simulink model "NearSpace_CMG_AttitudeValidation_S03_pitch45"  (R2024a)
settings: Solver=ode4  StartTime=0.0  StopTime=60  FixedStep=.001  RelTol=1e-3
InitFcn:
  | init_paths;
model workspace (MAT data in the model file):
  disturbance_schedule = [0 0.2 0.4 0.6 0.8 1 1.2 1.4 1.6 1.8 2 2.2 ... (1204 elements, 301x4)]
  native_controller_template : object (value not decoded)
  native_reference_bank : object (value not decoded)
  reference_attitude_deg = [0 0.2 0.4 0.6 0.8 1 1.2 1.4 1.6 1.8 2 2.2 ... (1204 elements, 301x4)]
  reference_body_rate = [0 0.2 0.4 0.6 0.8 1 1.2 1.4 1.6 1.8 2 2.2 ... (1204 elements, 301x4)]
  reference_torque_nom = [0 0.2 0.4 0.6 0.8 1 1.2 1.4 1.6 1.8 2 2.2 ... (1204 elements, 301x4)]
  reference_window = [-1e-06 0.199999 0.399999 0.599999 0.799999 0.999999 1.199999 1.399999 1.599999 1.799999 1.999999 2.199999 ... (130032 elements, 301x432)]
libraries: aerolibprivatev1p5 x1
(part 2 of 2)

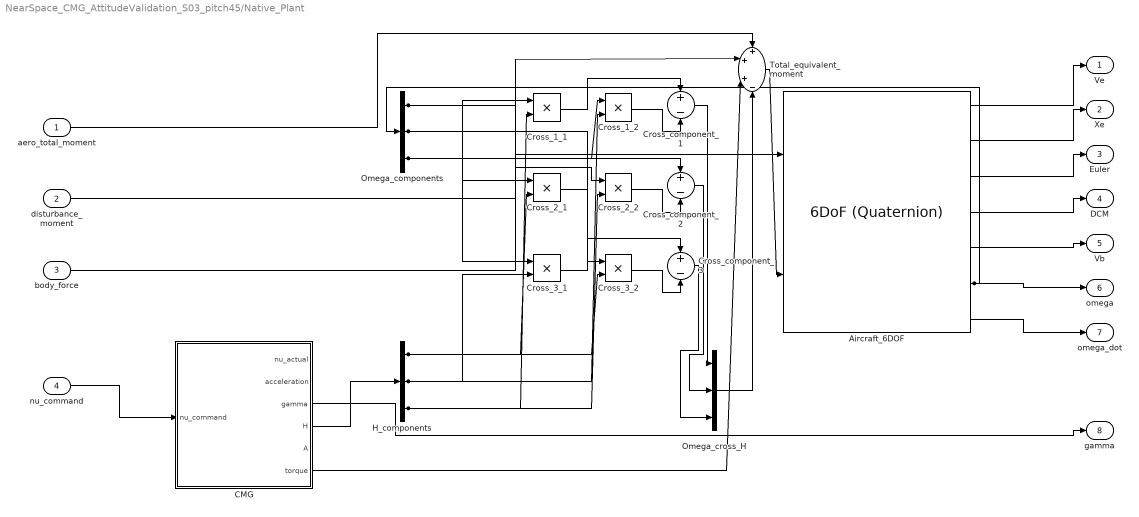
== system NearSpace_CMG_AttitudeValidation_S03_pitch45/Native_Plant ==
  aero_total_moment : Inport  PortDimensions=3
  disturbance_moment : Inport  Port=2  PortDimensions=3
  body_force : Inport  Port=3  PortDimensions=3
  nu_command : Inport  Port=4  PortDimensions=4
  Aircraft_6DOF : aerolibprivatev1p5/6DoF (Quaternion)  xme_0=[0 0 0]  Vm_0=[0 0 0]  eul_0=[-1.7740922954857791e-18;0.21106173041320209;0.087266462599716474]  pm_0=[0 -0.0043273206504133811 -6.9388939039072284e-15]  Mass=1200  Inertia=[1200 0 0;0 8500 0;0 0 9000]  k_quat=1.0
  CMG : Subsystem
  Cross_1_1 : Product
  Cross_1_2 : Product
  Cross_2_1 : Product
  Cross_2_2 : Product
  Cross_3_1 : Product
  Cross_3_2 : Product
  Cross_component_1 : Sum  Inputs=+-
  Cross_component_2 : Sum  Inputs=+-
  Cross_component_3 : Sum  Inputs=+-
  H_components : Demux  Outputs=3
  Omega_components : Demux  Outputs=3
  Omega_cross_H : Mux  Inputs=3
  Total_equivalent_moment : Sum  Inputs=+++-
  Ve : Outport
  Xe : Outport  Port=2
  Euler : Outport  Port=3
  DCM : Outport  Port=4
  Vb : Outport  Port=5
  omega : Outport  Port=6
  omega_dot : Outport  Port=7
  gamma : Outport  Port=8
  wires:
  nu_command/1 -> CMG/1(nu_command)
  Aircraft_6DOF/6 -> omega/1, Omega_components/1
  CMG/4(H) -> H_components/1
  Omega_components/2 -> Cross_3_2/1, Cross_1_1/1
  H_components/3 -> Cross_2_2/2, Cross_1_1/2
  Omega_components/3 -> Cross_2_1/1, Cross_1_2/1
  H_components/2 -> Cross_3_1/2, Cross_1_2/2
  Cross_1_1/1 -> Cross_component_1/1
  Cross_1_2/1 -> Cross_component_1/2
  H_components/1 -> Cross_3_2/2, Cross_2_1/2
  Omega_components/1 -> Cross_3_1/1, Cross_2_2/1
  Cross_2_1/1 -> Cross_component_2/1
  Cross_2_2/1 -> Cross_component_2/2
  Cross_3_1/1 -> Cross_component_3/1
  Cross_3_2/1 -> Cross_component_3/2
  Cross_component_1/1 -> Omega_cross_H/1
  Cross_component_2/1 -> Omega_cross_H/2
  Cross_component_3/1 -> Omega_cross_H/3
  aero_total_moment/1 -> Total_equivalent_moment/1
  disturbance_moment/1 -> Total_equivalent_moment/2
  CMG/6(torque) -> Total_equivalent_moment/3
  Omega_cross_H/1 -> Total_equivalent_moment/4
  Total_equivalent_moment/1 -> Aircraft_6DOF/2
  body_force/1 -> Aircraft_6DOF/1
  Aircraft_6DOF/1 -> Ve/1
  Aircraft_6DOF/2 -> Xe/1
  Aircraft_6DOF/3 -> Euler/1
  Aircraft_6DOF/4 -> DCM/1
  Aircraft_6DOF/5 -> Vb/1
  Aircraft_6DOF/7 -> omega_dot/1
  CMG/3(gamma) -> gamma/1

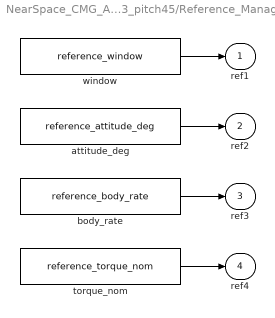
== system NearSpace_CMG_AttitudeValidation_S03_pitch45/Reference_Manager ==
  attitude_deg : FromWorkspace  VariableName=reference_attitude_deg  Interpolate=off  OutputAfterFinalValue=Holding final value
  body_rate : FromWorkspace  VariableName=reference_body_rate  Interpolate=off  OutputAfterFinalValue=Holding final value
  torque_nom : FromWorkspace  VariableName=reference_torque_nom  Interpolate=off  OutputAfterFinalValue=Holding final value
  window : FromWorkspace  VariableName=reference_window  Interpolate=off  OutputAfterFinalValue=Holding final value
  ref1 : Outport
  ref2 : Outport  Port=2
  ref3 : Outport  Port=3
  ref4 : Outport  Port=4
  wires:
  window/1 -> ref1/1
  attitude_deg/1 -> ref2/1
  body_rate/1 -> ref3/1
  torque_nom/1 -> ref4/1

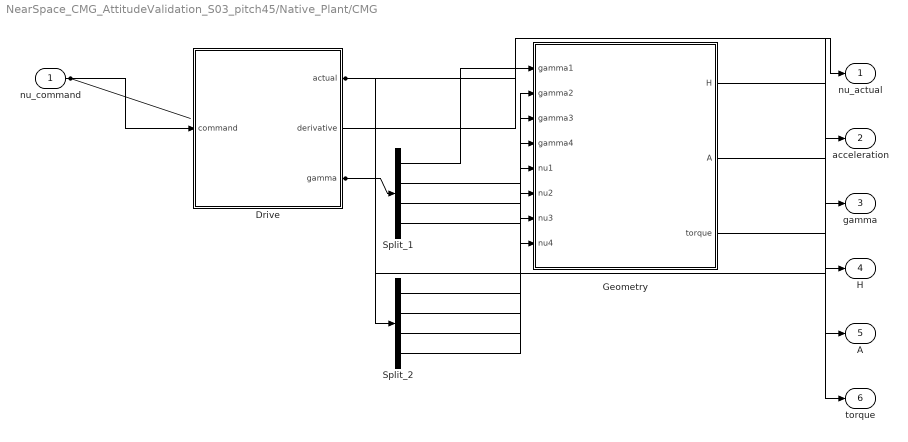
== system NearSpace_CMG_AttitudeValidation_S03_pitch45/Native_Plant/CMG ==
  nu_command : Inport  PortDimensions=4
  Drive : Subsystem
  Geometry : Subsystem
  Split_1 : Demux
  Split_2 : Demux
  nu_actual : Outport
  acceleration : Outport  Port=2
  gamma : Outport  Port=3
  H : Outport  Port=4
  A : Outport  Port=5
  torque : Outport  Port=6
  wires:
  Geometry/3(torque) -> torque/1
  Geometry/2(A) -> A/1
  Geometry/1(H) -> H/1
  Split_2/4 -> Geometry/8(nu4)
  Split_2/3 -> Geometry/7(nu3)
  Split_2/2 -> Geometry/6(nu2)
  Split_2/1 -> Geometry/5(nu1)
  Split_1/4 -> Geometry/4(gamma4)
  Split_1/3 -> Geometry/3(gamma3)
  Split_1/2 -> Geometry/2(gamma2)
  Split_1/1 -> Geometry/1(gamma1)
  nu_command/1 -> Drive/1(command)
  Drive/1(actual) -> Split_2/1, nu_actual/1
  Drive/2(derivative) -> acceleration/1
  Drive/3(gamma) -> Split_1/1, gamma/1

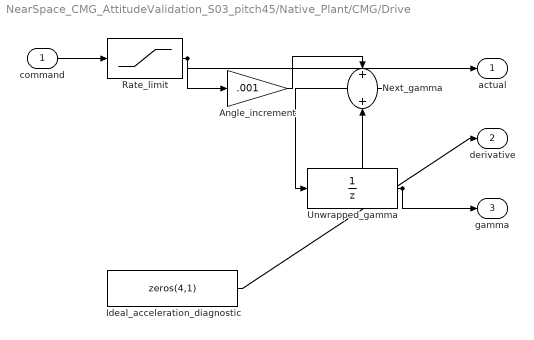
== system NearSpace_CMG_AttitudeValidation_S03_pitch45/Native_Plant/CMG/Drive ==
  command : Inport  PortDimensions=4
  Angle_increment : Gain  Gain=.001
  Ideal_acceleration_diagnostic : Constant  Value=zeros(4,1)
  Next_gamma : Sum
  Rate_limit : Saturate  UpperLimit=1  LowerLimit=-1
  Unwrapped_gamma : UnitDelay  InitialCondition=[0 0 0 0]  SampleTime=.001
  actual : Outport
  derivative : Outport  Port=2
  gamma : Outport  Port=3
  wires:
  command/1 -> Rate_limit/1
  Rate_limit/1 -> actual/1, Angle_increment/1
  Angle_increment/1 -> Next_gamma/1
  Unwrapped_gamma/1 -> Next_gamma/2, gamma/1
  Next_gamma/1 -> Unwrapped_gamma/1
  Ideal_acceleration_diagnostic/1 -> derivative/1

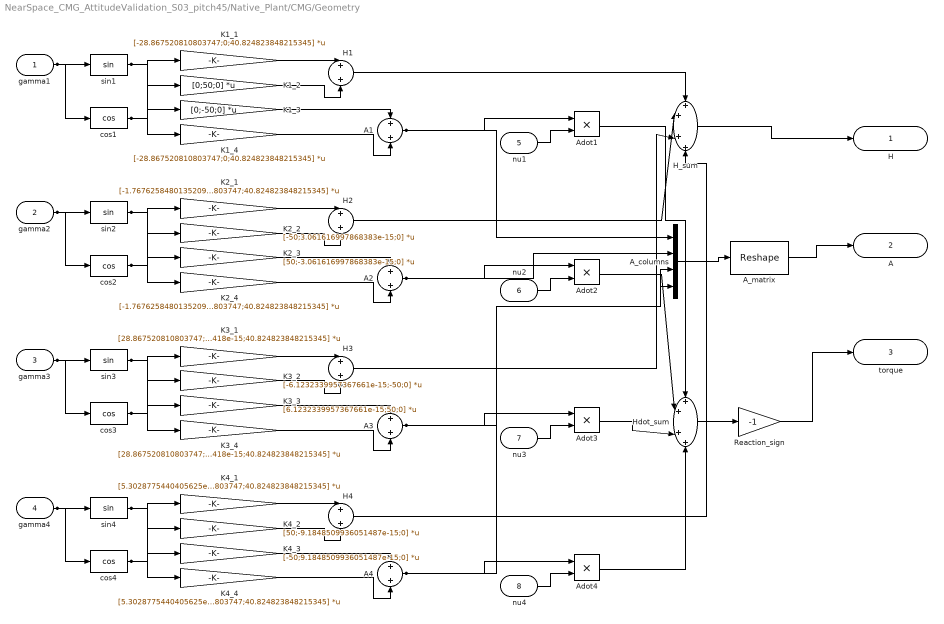
== system NearSpace_CMG_AttitudeValidation_S03_pitch45/Native_Plant/CMG/Geometry ==
  gamma1 : Inport
  gamma2 : Inport  Port=2
  gamma3 : Inport  Port=3
  gamma4 : Inport  Port=4
  nu1 : Inport  Port=5
  nu2 : Inport  Port=6
  nu3 : Inport  Port=7
  nu4 : Inport  Port=8
  A{1..4} (4 alike) : Sum
  A_columns : Mux
  A_matrix : Reshape  OutputDimensionality=Customize  OutputDimensions=[3 4]
  Adot{1..4} (4 alike) : Product
  H{1..4} (4 alike) : Sum
  H_sum : Sum  Inputs=++++
  Hdot_sum : Sum  Inputs=++++
  K1_1 : Gain  Gain=[-28.867520810803747;0;40.824823848215345]  Multiplication=Matrix(K*u)
  K1_2 : Gain  Gain=[0;50;0]  Multiplication=Matrix(K*u)
  K1_3 : Gain  Gain=[0;-50;0]  Multiplication=Matrix(K*u)
  K1_4 : Gain  Gain=[-28.867520810803747;0;40.824823848215345]  Multiplication=Matrix(K*u)
  K2_1 : Gain  Gain=[-1.7676258480135209e-15;-28.867520810803747;40.824823848215345]  Multiplication=Matrix(K*u)
  K2_2 : Gain  Gain=[-50;3.061616997868383e-15;0]  Multiplication=Matrix(K*u)
  K2_3 : Gain  Gain=[50;-3.061616997868383e-15;0]  Multiplication=Matrix(K*u)
  K2_4 : Gain  Gain=[-1.7676258480135209e-15;-28.867520810803747;40.824823848215345]  Multiplication=Matrix(K*u)
  K3_1 : Gain  Gain=[28.867520810803747;-3.5352516960270418e-15;40.824823848215345]  Multiplication=Matrix(K*u)
  K3_2 : Gain  Gain=[-6.1232339957367661e-15;-50;0]  Multiplication=Matrix(K*u)
  K3_3 : Gain  Gain=[6.1232339957367661e-15;50;0]  Multiplication=Matrix(K*u)
  K3_4 : Gain  Gain=[28.867520810803747;-3.5352516960270418e-15;40.824823848215345]  Multiplication=Matrix(K*u)
  K4_1 : Gain  Gain=[5.3028775440405625e-15;28.867520810803747;40.824823848215345]  Multiplication=Matrix(K*u)
  K4_2 : Gain  Gain=[50;-9.1848509936051487e-15;0]  Multiplication=Matrix(K*u)
  K4_3 : Gain  Gain=[-50;9.1848509936051487e-15;0]  Multiplication=Matrix(K*u)
  K4_4 : Gain  Gain=[5.3028775440405625e-15;28.867520810803747;40.824823848215345]  Multiplication=Matrix(K*u)
  Reaction_sign : Gain  Gain=-1
  cos{1..4} (4 alike) : Trigonometry  Operator=cos
  sin{1..4} (4 alike) : Trigonometry
  H : Outport
  A : Outport  Port=2
  torque : Outport  Port=3
  wires:
  sin1/1 -> K1_3/1, K1_1/1
  cos1/1 -> K1_4/1, K1_2/1
  K1_1/1 -> H1/1
  K1_2/1 -> H1/2
  K1_3/1 -> A1/1
  K1_4/1 -> A1/2
  A1/1 -> A_columns/1, Adot1/1
  sin2/1 -> K2_3/1, K2_1/1
  cos2/1 -> K2_4/1, K2_2/1
  K2_1/1 -> H2/1
  K2_2/1 -> H2/2
  K2_3/1 -> A2/1
  K2_4/1 -> A2/2
  A2/1 -> A_columns/2, Adot2/1
  sin3/1 -> K3_3/1, K3_1/1
  cos3/1 -> K3_4/1, K3_2/1
  K3_1/1 -> H3/1
  K3_2/1 -> H3/2
  K3_3/1 -> A3/1
  K3_4/1 -> A3/2
  A3/1 -> A_columns/3, Adot3/1
  sin4/1 -> K4_3/1, K4_1/1
  cos4/1 -> K4_4/1, K4_2/1
  K4_1/1 -> H4/1
  K4_2/1 -> H4/2
  K4_3/1 -> A4/1
  K4_4/1 -> A4/2
  A4/1 -> A_columns/4, Adot4/1
  H1/1 -> H_sum/1
  Adot1/1 -> Hdot_sum/1
  H2/1 -> H_sum/2
  Adot2/1 -> Hdot_sum/2
  H3/1 -> H_sum/3
  Adot3/1 -> Hdot_sum/3
  H4/1 -> H_sum/4
  Adot4/1 -> Hdot_sum/4
  A_columns/1 -> A_matrix/1
  Hdot_sum/1 -> Reaction_sign/1
  gamma1/1 -> cos1/1, sin1/1
  nu1/1 -> Adot1/2
  gamma2/1 -> cos2/1, sin2/1
  nu2/1 -> Adot2/2
  gamma3/1 -> cos3/1, sin3/1
  nu3/1 -> Adot3/2
  gamma4/1 -> cos4/1, sin4/1
  nu4/1 -> Adot4/2
  H_sum/1 -> H/1
  A_matrix/1 -> A/1
  Reaction_sign/1 -> torque/1
